simulink library "Contact_Forces_Lib"  (R2025a)
settings: Solver=ode45  StartTime=0.0  StopTime=10.0  RelTol=1e-3  EnableMultiTasking=on
undefined symbols (not defined in the file or in its folder): b_contact, custom_param_1, custom_param_2, Extr_Data_Ring, k_contact, l_cone, length_cylinder, length_tube, mu_kinetic, mu_static, pen_exponent, pen_full_damp_F, rad_s_cone, radius_cylinder, radius_tube, v_thr, X, Y, Z
libraries: nesl_utility x197, sm_lib x115, $bdroot x72, simulink x20, fl_lib x4
(part 9 of 12)

== system Contact_Forces_Lib/2D/Composite Forces/Box to Box Force/BoxB Corners ==
  Circle to Line C1 AC : $bdroot/2D/Circle to Finite Line Force  circle_rad=boxB_contact_rad  line_depth=boxF_h/2  line_length=boxF_l  force_law=Linear  k_contact=k_contact_box2box  b_contact=b_contact_box2box  pen_full_damp_F=pen_full_damp_F_box2box  pen_exponent=pen_exponent_box2box  custom_param_1=1  custom_param_2=1  friction_law=None  mu_kinetic=mu_kinetic_box2box  mu_static=mu_static_box2box  v_thr=v_thr_box2box  vis_on=off  vis_opc_en=0  vis_len_linBz=vis_len_boxFz  vis_len_linBx=vis_len_boxFx  vis_len_cirFz=vis_len_boxBz  vis_len_cirFx=vis_len_boxBx  vis_clr=vis_clr_box2box  vis_opc=vis_opc_box2box
  Circle to Line C1 BD : $bdroot/2D/Circle to Finite Line Force  circle_rad=boxB_contact_rad  line_depth=boxF_l/2  line_length=boxF_h  force_law=Linear  k_contact=k_contact_box2box  b_contact=b_contact_box2box  pen_full_damp_F=pen_full_damp_F_box2box  pen_exponent=pen_exponent_box2box  custom_param_1=1  custom_param_2=1  friction_law=None  mu_kinetic=mu_kinetic_box2box  mu_static=mu_static_box2box  v_thr=v_thr_box2box  vis_on=off  vis_opc_en=0  vis_len_linBz=vis_len_boxFz  vis_len_linBx=vis_len_boxFx  vis_len_cirFz=vis_len_boxBz  vis_len_cirFx=vis_len_boxBx  vis_clr=vis_clr_box2box  vis_opc=vis_opc_box2box
  Circle to Line C2 AC : $bdroot/2D/Circle to Finite Line Force  circle_rad=boxB_contact_rad  line_depth=boxF_h/2  line_length=boxF_l  force_law=Linear  k_contact=k_contact_box2box  b_contact=b_contact_box2box  pen_full_damp_F=pen_full_damp_F_box2box  pen_exponent=pen_exponent_box2box  custom_param_1=1  custom_param_2=1  friction_law=None  mu_kinetic=mu_kinetic_box2box  mu_static=mu_static_box2box  v_thr=v_thr_box2box  vis_on=off  vis_opc_en=0  vis_len_linBz=vis_len_boxFz  vis_len_linBx=vis_len_boxFx  vis_len_cirFz=vis_len_boxBz  vis_len_cirFx=vis_len_boxBx  vis_clr=vis_clr_box2box  vis_opc=vis_opc_box2box
  Circle to Line C2 BD : $bdroot/2D/Circle to Finite Line Force  circle_rad=boxB_contact_rad  line_depth=boxF_l/2  line_length=boxF_h  force_law=Linear  k_contact=k_contact_box2box  b_contact=b_contact_box2box  pen_full_damp_F=pen_full_damp_F_box2box  pen_exponent=pen_exponent_box2box  custom_param_1=1  custom_param_2=1  friction_law=None  mu_kinetic=mu_kinetic_box2box  mu_static=mu_static_box2box  v_thr=v_thr_box2box  vis_on=off  vis_opc_en=0  vis_len_linBz=vis_len_boxFz  vis_len_linBx=vis_len_boxFx  vis_len_cirFz=vis_len_boxBz  vis_len_cirFx=vis_len_boxBx  vis_clr=vis_clr_box2box  vis_opc=vis_opc_box2box
  Circle to Line C3 AC : $bdroot/2D/Circle to Finite Line Force  circle_rad=boxB_contact_rad  line_depth=boxF_h/2  line_length=boxF_l  force_law=Linear  k_contact=k_contact_box2box  b_contact=b_contact_box2box  pen_full_damp_F=pen_full_damp_F_box2box  pen_exponent=pen_exponent_box2box  custom_param_1=1  custom_param_2=1  friction_law=None  mu_kinetic=mu_kinetic_box2box  mu_static=mu_static_box2box  v_thr=v_thr_box2box  vis_on=off  vis_opc_en=0  vis_len_linBz=vis_len_boxFz  vis_len_linBx=vis_len_boxFx  vis_len_cirFz=vis_len_boxBz  vis_len_cirFx=vis_len_boxBx  vis_clr=vis_clr_box2box  vis_opc=vis_opc_box2box
  Circle to Line C3 BD : $bdroot/2D/Circle to Finite Line Force  circle_rad=boxB_contact_rad  line_depth=boxF_l/2  line_length=boxF_h  force_law=Linear  k_contact=k_contact_box2box  b_contact=b_contact_box2box  pen_full_damp_F=pen_full_damp_F_box2box  pen_exponent=pen_exponent_box2box  custom_param_1=1  custom_param_2=1  friction_law=None  mu_kinetic=mu_kinetic_box2box  mu_static=mu_static_box2box  v_thr=v_thr_box2box  vis_on=off  vis_opc_en=0  vis_len_linBz=vis_len_boxFz  vis_len_linBx=vis_len_boxFx  vis_len_cirFz=vis_len_boxBz  vis_len_cirFx=vis_len_boxBx  vis_clr=vis_clr_box2box  vis_opc=vis_opc_box2box
  Circle to Line C4 AC : $bdroot/2D/Circle to Finite Line Force  circle_rad=boxB_contact_rad  line_depth=boxF_h/2  line_length=boxF_l  force_law=Linear  k_contact=k_contact_box2box  b_contact=b_contact_box2box  pen_full_damp_F=pen_full_damp_F_box2box  pen_exponent=pen_exponent_box2box  custom_param_1=1  custom_param_2=1  friction_law=None  mu_kinetic=mu_kinetic_box2box  mu_static=mu_static_box2box  v_thr=v_thr_box2box  vis_on=off  vis_opc_en=0  vis_len_linBz=vis_len_boxFz  vis_len_linBx=vis_len_boxFx  vis_len_cirFz=vis_len_boxBz  vis_len_cirFx=vis_len_boxBx  vis_clr=vis_clr_box2box  vis_opc=vis_opc_box2box
  Circle to Line C4 BD : $bdroot/2D/Circle to Finite Line Force  circle_rad=boxB_contact_rad  line_depth=boxF_l/2  line_length=boxF_h  force_law=Linear  k_contact=k_contact_box2box  b_contact=b_contact_box2box  pen_full_damp_F=pen_full_damp_F_box2box  pen_exponent=pen_exponent_box2box  custom_param_1=1  custom_param_2=1  friction_law=None  mu_kinetic=mu_kinetic_box2box  mu_static=mu_static_box2box  v_thr=v_thr_box2box  vis_on=off  vis_opc_en=0  vis_len_linBz=vis_len_boxFz  vis_len_linBx=vis_len_boxFx  vis_len_cirFz=vis_len_boxBz  vis_len_cirFx=vis_len_boxBx  vis_clr=vis_clr_box2box  vis_opc=vis_opc_box2box
  Forces : Subsystem
  Transform  C1 : sm_lib/Frames and Transforms/Rigid Transform  RotationMethod=None  FollAlignAxisA=+X  BaseAlignAxisA=+Y  FollAlignAxisB=+Y  BaseAlignAxisB=+Z  RotationStandardAxis=+Z  RotationAngle=0  RotationAngleUnits=deg  RotationArbitraryAxis=[0 0 1]  RotationSequenceAxes=FollowerAxes  RotationSequence=XYX  RotationSequenceAngles=[0 0 0]  RotationSequenceAnglesUnits=deg  RotationMatrix=[1 0 0; 0 1 0; 0 0 1]  Quaternion=[1 0 0 0]  TranslationMethod=Cartesian  TranslationCartesianOffset=[-(boxB_h/2-boxB_contact_rad) -(boxB_l/2-boxB_contact_rad) 0]  TranslationCartesianOffsetUnits=m  TranslationStandardAxis=+Y  TranslationStandardOffset=0.1  TranslationStandardOffsetUnits=m  TranslationROffset=0  TranslationROffsetUnits=m  TranslationThetaOffset=0  TranslationThetaOffsetUnits=deg  TranslationZOffset=0  TranslationZOffsetUnits=m
  Transform  C2 : sm_lib/Frames and Transforms/Rigid Transform  RotationMethod=None  FollAlignAxisA=+X  BaseAlignAxisA=+Y  FollAlignAxisB=+Y  BaseAlignAxisB=+Z  RotationStandardAxis=+Z  RotationAngle=0  RotationAngleUnits=deg  RotationArbitraryAxis=[0 0 1]  RotationSequenceAxes=FollowerAxes  RotationSequence=XYX  RotationSequenceAngles=[0 0 0]  RotationSequenceAnglesUnits=deg  RotationMatrix=[1 0 0; 0 1 0; 0 0 1]  Quaternion=[1 0 0 0]  TranslationMethod=Cartesian  TranslationCartesianOffset=[-(boxB_h/2-boxB_contact_rad) (boxB_l/2-boxB_contact_rad) 0]  TranslationCartesianOffsetUnits=m  TranslationStandardAxis=+Y  TranslationStandardOffset=0.1  TranslationStandardOffsetUnits=m  TranslationROffset=0  TranslationROffsetUnits=m  TranslationThetaOffset=0  TranslationThetaOffsetUnits=deg  TranslationZOffset=0  TranslationZOffsetUnits=m
  Transform  C3 : sm_lib/Frames and Transforms/Rigid Transform  RotationMethod=None  FollAlignAxisA=+X  BaseAlignAxisA=+Y  FollAlignAxisB=+Y  BaseAlignAxisB=+Z  RotationStandardAxis=+Z  RotationAngle=0  RotationAngleUnits=deg  RotationArbitraryAxis=[0 0 1]  RotationSequenceAxes=FollowerAxes  RotationSequence=XYX  RotationSequenceAngles=[0 0 0]  RotationSequenceAnglesUnits=deg  RotationMatrix=[1 0 0; 0 1 0; 0 0 1]  Quaternion=[1 0 0 0]  TranslationMethod=Cartesian  TranslationCartesianOffset=[(boxB_h/2-boxB_contact_rad) (boxB_l/2-boxB_contact_rad) 0]  TranslationCartesianOffsetUnits=m  TranslationStandardAxis=+Y  TranslationStandardOffset=0.1  TranslationStandardOffsetUnits=m  TranslationROffset=0  TranslationROffsetUnits=m  TranslationThetaOffset=0  TranslationThetaOffsetUnits=deg  TranslationZOffset=0  TranslationZOffsetUnits=m
  Transform  C4 : sm_lib/Frames and Transforms/Rigid Transform  RotationMethod=None  FollAlignAxisA=+X  BaseAlignAxisA=+Y  FollAlignAxisB=+Y  BaseAlignAxisB=+Z  RotationStandardAxis=+Z  RotationAngle=0  RotationAngleUnits=deg  RotationArbitraryAxis=[0 0 1]  RotationSequenceAxes=FollowerAxes  RotationSequence=XYX  RotationSequenceAngles=[0 0 0]  RotationSequenceAnglesUnits=deg  RotationMatrix=[1 0 0; 0 1 0; 0 0 1]  Quaternion=[1 0 0 0]  TranslationMethod=Cartesian  TranslationCartesianOffset=[(boxB_h/2-boxB_contact_rad) -(boxB_l/2-boxB_contact_rad) 0]  TranslationCartesianOffsetUnits=m  TranslationStandardAxis=+Y  TranslationStandardOffset=0.1  TranslationStandardOffsetUnits=m  TranslationROffset=0  TranslationROffsetUnits=m  TranslationThetaOffset=0  TranslationThetaOffsetUnits=deg  TranslationZOffset=0  TranslationZOffsetUnits=m
  Transform BD : sm_lib/Frames and Transforms/Rigid Transform  RotationMethod=StandardAxis  FollAlignAxisA=+X  BaseAlignAxisA=+Y  FollAlignAxisB=+Y  BaseAlignAxisB=+Z  RotationStandardAxis=+Z  RotationAngle=90  RotationAngleUnits=deg  RotationArbitraryAxis=[0 0 1]  RotationSequenceAxes=FollowerAxes  RotationSequence=XYX  RotationSequenceAngles=[0 0 0]  RotationSequenceAnglesUnits=deg  RotationMatrix=[1 0 0; 0 1 0; 0 0 1]  Quaternion=[1 0 0 0]  TranslationMethod=None  TranslationCartesianOffset=[0 0 0]  TranslationCartesianOffsetUnits=m  TranslationStandardAxis=+Y  TranslationStandardOffset=0.1  TranslationStandardOffsetUnits=m  TranslationROffset=0  TranslationROffsetUnits=m  TranslationThetaOffset=0  TranslationThetaOffsetUnits=deg  TranslationZOffset=0  TranslationZOffsetUnits=m
  BoxB : PMIOPort  Side=Left
  BoxF : PMIOPort  Port=2  Side=Right
  wires:
  Circle to Line C4 BD/1 -> Forces/8(4BD)
  Circle to Line C2 BD/1 -> Forces/4(2BD)
  Circle to Line C3 BD/1 -> Forces/6(3BD)
  Circle to Line C1 AC/1 -> Forces/1(1AC)
  Circle to Line C3 AC/1 -> Forces/5(3AC)
  Circle to Line C4 AC/1 -> Forces/7(4AC)
  Circle to Line C2 AC/1 -> Forces/3(2AC)
  Circle to Line C1 BD/1 -> Forces/2(1BD)
  connections:
  Circle to Line C3 BD/RConn1 -- Circle to Line C4 BD/RConn1 -- Circle to Line C2 BD/RConn1 -- Transform BD/RConn1 -- Circle to Line C1 BD/RConn1
  Circle to Line C1 AC/LConn1 -- Circle to Line C1 BD/LConn1 -- Transform  C1/RConn1
  Transform BD/LConn1 -- BoxF/RConn1 -- Circle to Line C3 AC/RConn1 -- Circle to Line C4 AC/RConn1 -- Circle to Line C2 AC/RConn1 -- Circle to Line C1 AC/RConn1
  Transform  C3/LConn1 -- Transform  C4/LConn1 -- BoxB/RConn1 -- Transform  C1/LConn1 -- Transform  C2/LConn1
  Circle to Line C3 AC/LConn1 -- Circle to Line C3 BD/LConn1 -- Transform  C3/RConn1
  Circle to Line C4 AC/LConn1 -- Circle to Line C4 BD/LConn1 -- Transform  C4/RConn1
  Circle to Line C2 AC/LConn1 -- Circle to Line C2 BD/LConn1 -- Transform  C2/RConn1

== system Contact_Forces_Lib/2D/Composite Forces/Box to Box Force/BoxF Corners ==
  Circle to Line C1 AC : $bdroot/2D/Circle to Finite Line Force  circle_rad=boxF_contact_rad  line_depth=boxB_h/2  line_length=boxB_l  force_law=Linear  k_contact=k_contact_box2box  b_contact=b_contact_box2box  pen_full_damp_F=pen_full_damp_F_box2box  pen_exponent=pen_exponent_box2box  custom_param_1=1  custom_param_2=1  friction_law=None  mu_kinetic=mu_kinetic_box2box  mu_static=mu_static_box2box  v_thr=v_thr_box2box  vis_on=off  vis_opc_en=0  vis_len_linBz=vis_len_boxBz  vis_len_linBx=vis_len_boxBx  vis_len_cirFz=vis_len_boxFz  vis_len_cirFx=vis_len_boxFx  vis_clr=vis_clr_box2box  vis_opc=vis_opc_box2box
  Circle to Line C1 BD : $bdroot/2D/Circle to Finite Line Force  circle_rad=boxF_contact_rad  line_depth=boxB_l/2  line_length=boxB_h  force_law=Linear  k_contact=k_contact_box2box  b_contact=b_contact_box2box  pen_full_damp_F=pen_full_damp_F_box2box  pen_exponent=pen_exponent_box2box  custom_param_1=1  custom_param_2=1  friction_law=None  mu_kinetic=mu_kinetic_box2box  mu_static=mu_static_box2box  v_thr=v_thr_box2box  vis_on=off  vis_opc_en=0  vis_len_linBz=vis_len_boxBz  vis_len_linBx=vis_len_boxBx  vis_len_cirFz=vis_len_boxFz  vis_len_cirFx=vis_len_boxFx  vis_clr=vis_clr_box2box  vis_opc=vis_opc_box2box
  Circle to Line C2 AC : $bdroot/2D/Circle to Finite Line Force  circle_rad=boxF_contact_rad  line_depth=boxB_h/2  line_length=boxB_l  force_law=Linear  k_contact=k_contact_box2box  b_contact=b_contact_box2box  pen_full_damp_F=pen_full_damp_F_box2box  pen_exponent=pen_exponent_box2box  custom_param_1=1  custom_param_2=1  friction_law=None  mu_kinetic=mu_kinetic_box2box  mu_static=mu_static_box2box  v_thr=v_thr_box2box  vis_on=off  vis_opc_en=0  vis_len_linBz=vis_len_boxBz  vis_len_linBx=vis_len_boxBx  vis_len_cirFz=vis_len_boxFz  vis_len_cirFx=vis_len_boxFx  vis_clr=vis_clr_box2box  vis_opc=vis_opc_box2box
  Circle to Line C2 BD : $bdroot/2D/Circle to Finite Line Force  circle_rad=boxF_contact_rad  line_depth=boxB_l/2  line_length=boxB_h  force_law=Linear  k_contact=k_contact_box2box  b_contact=b_contact_box2box  pen_full_damp_F=pen_full_damp_F_box2box  pen_exponent=pen_exponent_box2box  custom_param_1=1  custom_param_2=1  friction_law=None  mu_kinetic=mu_kinetic_box2box  mu_static=mu_static_box2box  v_thr=v_thr_box2box  vis_on=off  vis_opc_en=0  vis_len_linBz=vis_len_boxBz  vis_len_linBx=vis_len_boxBx  vis_len_cirFz=vis_len_boxFz  vis_len_cirFx=vis_len_boxFx  vis_clr=vis_clr_box2box  vis_opc=vis_opc_box2box
  Circle to Line C3 AC : $bdroot/2D/Circle to Finite Line Force  circle_rad=boxF_contact_rad  line_depth=boxB_h/2  line_length=boxB_l  force_law=Linear  k_contact=k_contact_box2box  b_contact=b_contact_box2box  pen_full_damp_F=pen_full_damp_F_box2box  pen_exponent=pen_exponent_box2box  custom_param_1=1  custom_param_2=1  friction_law=None  mu_kinetic=mu_kinetic_box2box  mu_static=mu_static_box2box  v_thr=v_thr_box2box  vis_on=off  vis_opc_en=0  vis_len_linBz=vis_len_boxBz  vis_len_linBx=vis_len_boxBx  vis_len_cirFz=vis_len_boxFz  vis_len_cirFx=vis_len_boxFx  vis_clr=vis_clr_box2box  vis_opc=vis_opc_box2box
  Circle to Line C3 BD : $bdroot/2D/Circle to Finite Line Force  circle_rad=boxF_contact_rad  line_depth=boxB_l/2  line_length=boxB_h  force_law=Linear  k_contact=k_contact_box2box  b_contact=b_contact_box2box  pen_full_damp_F=pen_full_damp_F_box2box  pen_exponent=pen_exponent_box2box  custom_param_1=1  custom_param_2=1  friction_law=None  mu_kinetic=mu_kinetic_box2box  mu_static=mu_static_box2box  v_thr=v_thr_box2box  vis_on=off  vis_opc_en=0  vis_len_linBz=vis_len_boxBz  vis_len_linBx=vis_len_boxBx  vis_len_cirFz=vis_len_boxFz  vis_len_cirFx=vis_len_boxFx  vis_clr=vis_clr_box2box  vis_opc=vis_opc_box2box
  Circle to Line C4 AC : $bdroot/2D/Circle to Finite Line Force  circle_rad=boxF_contact_rad  line_depth=boxB_h/2  line_length=boxB_l  force_law=Linear  k_contact=k_contact_box2box  b_contact=b_contact_box2box  pen_full_damp_F=pen_full_damp_F_box2box  pen_exponent=pen_exponent_box2box  custom_param_1=1  custom_param_2=1  friction_law=None  mu_kinetic=mu_kinetic_box2box  mu_static=mu_static_box2box  v_thr=v_thr_box2box  vis_on=off  vis_opc_en=0  vis_len_linBz=vis_len_boxBz  vis_len_linBx=vis_len_boxBx  vis_len_cirFz=vis_len_boxFz  vis_len_cirFx=vis_len_boxFx  vis_clr=vis_clr_box2box  vis_opc=vis_opc_box2box
  Circle to Line C4 BD : $bdroot/2D/Circle to Finite Line Force  circle_rad=boxF_contact_rad  line_depth=boxB_l/2  line_length=boxB_h  force_law=Linear  k_contact=k_contact_box2box  b_contact=b_contact_box2box  pen_full_damp_F=pen_full_damp_F_box2box  pen_exponent=pen_exponent_box2box  custom_param_1=1  custom_param_2=1  friction_law=None  mu_kinetic=mu_kinetic_box2box  mu_static=mu_static_box2box  v_thr=v_thr_box2box  vis_on=off  vis_opc_en=0  vis_len_linBz=vis_len_boxBz  vis_len_linBx=vis_len_boxBx  vis_len_cirFz=vis_len_boxFz  vis_len_cirFx=vis_len_boxFx  vis_clr=vis_clr_box2box  vis_opc=vis_opc_box2box
  Forces : Subsystem
  Transform BD : sm_lib/Frames and Transforms/Rigid Transform  RotationMethod=StandardAxis  FollAlignAxisA=+X  BaseAlignAxisA=+Y  FollAlignAxisB=+Y  BaseAlignAxisB=+Z  RotationStandardAxis=+Z  RotationAngle=90  RotationAngleUnits=deg  RotationArbitraryAxis=[0 0 1]  RotationSequenceAxes=FollowerAxes  RotationSequence=XYX  RotationSequenceAngles=[0 0 0]  RotationSequenceAnglesUnits=deg  RotationMatrix=[1 0 0; 0 1 0; 0 0 1]  Quaternion=[1 0 0 0]  TranslationMethod=None  TranslationCartesianOffset=[0 0 0]  TranslationCartesianOffsetUnits=m  TranslationStandardAxis=+Y  TranslationStandardOffset=0.1  TranslationStandardOffsetUnits=m  TranslationROffset=0  TranslationROffsetUnits=m  TranslationThetaOffset=0  TranslationThetaOffsetUnits=deg  TranslationZOffset=0  TranslationZOffsetUnits=m
  Transform C1 : sm_lib/Frames and Transforms/Rigid Transform  RotationMethod=None  FollAlignAxisA=+X  BaseAlignAxisA=+Y  FollAlignAxisB=+Y  BaseAlignAxisB=+Z  RotationStandardAxis=+Z  RotationAngle=0  RotationAngleUnits=deg  RotationArbitraryAxis=[0 0 1]  RotationSequenceAxes=FollowerAxes  RotationSequence=XYX  RotationSequenceAngles=[0 0 0]  RotationSequenceAnglesUnits=deg  RotationMatrix=[1 0 0; 0 1 0; 0 0 1]  Quaternion=[1 0 0 0]  TranslationMethod=Cartesian  TranslationCartesianOffset=[-(boxF_h/2-boxF_contact_rad) -(boxF_l/2-boxF_contact_rad) 0]  TranslationCartesianOffsetUnits=m  TranslationStandardAxis=+Y  TranslationStandardOffset=0.1  TranslationStandardOffsetUnits=m  TranslationROffset=0  TranslationROffsetUnits=m  TranslationThetaOffset=0  TranslationThetaOffsetUnits=deg  TranslationZOffset=0  TranslationZOffsetUnits=m
  Transform C2 : sm_lib/Frames and Transforms/Rigid Transform  RotationMethod=None  FollAlignAxisA=+X  BaseAlignAxisA=+Y  FollAlignAxisB=+Y  BaseAlignAxisB=+Z  RotationStandardAxis=+Z  RotationAngle=0  RotationAngleUnits=deg  RotationArbitraryAxis=[0 0 1]  RotationSequenceAxes=FollowerAxes  RotationSequence=XYX  RotationSequenceAngles=[0 0 0]  RotationSequenceAnglesUnits=deg  RotationMatrix=[1 0 0; 0 1 0; 0 0 1]  Quaternion=[1 0 0 0]  TranslationMethod=Cartesian  TranslationCartesianOffset=[-(boxF_h/2-boxF_contact_rad) (boxF_l/2-boxF_contact_rad) 0]  TranslationCartesianOffsetUnits=m  TranslationStandardAxis=+Y  TranslationStandardOffset=0.1  TranslationStandardOffsetUnits=m  TranslationROffset=0  TranslationROffsetUnits=m  TranslationThetaOffset=0  TranslationThetaOffsetUnits=deg  TranslationZOffset=0  TranslationZOffsetUnits=m
  Transform C3 : sm_lib/Frames and Transforms/Rigid Transform  RotationMethod=None  FollAlignAxisA=+X  BaseAlignAxisA=+Y  FollAlignAxisB=+Y  BaseAlignAxisB=+Z  RotationStandardAxis=+Z  RotationAngle=0  RotationAngleUnits=deg  RotationArbitraryAxis=[0 0 1]  RotationSequenceAxes=FollowerAxes  RotationSequence=XYX  RotationSequenceAngles=[0 0 0]  RotationSequenceAnglesUnits=deg  RotationMatrix=[1 0 0; 0 1 0; 0 0 1]  Quaternion=[1 0 0 0]  TranslationMethod=Cartesian  TranslationCartesianOffset=[(boxF_h/2-boxF_contact_rad) (boxF_l/2-boxF_contact_rad) 0]  TranslationCartesianOffsetUnits=m  TranslationStandardAxis=+Y  TranslationStandardOffset=0.1  TranslationStandardOffsetUnits=m  TranslationROffset=0  TranslationROffsetUnits=m  TranslationThetaOffset=0  TranslationThetaOffsetUnits=deg  TranslationZOffset=0  TranslationZOffsetUnits=m
  Transform C4 : sm_lib/Frames and Transforms/Rigid Transform  RotationMethod=None  FollAlignAxisA=+X  BaseAlignAxisA=+Y  FollAlignAxisB=+Y  BaseAlignAxisB=+Z  RotationStandardAxis=+Z  RotationAngle=0  RotationAngleUnits=deg  RotationArbitraryAxis=[0 0 1]  RotationSequenceAxes=FollowerAxes  RotationSequence=XYX  RotationSequenceAngles=[0 0 0]  RotationSequenceAnglesUnits=deg  RotationMatrix=[1 0 0; 0 1 0; 0 0 1]  Quaternion=[1 0 0 0]  TranslationMethod=Cartesian  TranslationCartesianOffset=[(boxF_h/2-boxF_contact_rad) -(boxF_l/2-boxF_contact_rad) 0]  TranslationCartesianOffsetUnits=m  TranslationStandardAxis=+Y  TranslationStandardOffset=0.1  TranslationStandardOffsetUnits=m  TranslationROffset=0  TranslationROffsetUnits=m  TranslationThetaOffset=0  TranslationThetaOffsetUnits=deg  TranslationZOffset=0  TranslationZOffsetUnits=m
  BoxB : PMIOPort  Side=Left
  BoxF : PMIOPort  Port=2  Side=Right
  wires:
  Circle to Line C4 AC/1 -> Forces/7(4AC)
  Circle to Line C1 BD/1 -> Forces/2(1BD)
  Circle to Line C2 AC/1 -> Forces/3(2AC)
  Circle to Line C3 BD/1 -> Forces/6(3BD)
  Circle to Line C4 BD/1 -> Forces/8(4BD)
  Circle to Line C2 BD/1 -> Forces/4(2BD)
  Circle to Line C3 AC/1 -> Forces/5(3AC)
  Circle to Line C1 AC/1 -> Forces/1(1AC)
  connections:
  Circle to Line C1 BD/RConn1 -- Transform BD/RConn1 -- Circle to Line C3 BD/RConn1 -- Circle to Line C4 BD/RConn1 -- Circle to Line C2 BD/RConn1
  Circle to Line C2 AC/LConn1 -- Circle to Line C2 BD/LConn1 -- Transform C2/RConn1
  Circle to Line C3 AC/LConn1 -- Circle to Line C3 BD/LConn1 -- Transform C3/RConn1
  Transform C3/LConn1 -- Transform C4/LConn1 -- Transform C1/LConn1 -- Transform C2/LConn1 -- BoxF/RConn1
  Circle to Line C4 AC/LConn1 -- Circle to Line C4 BD/LConn1 -- Transform C4/RConn1
  Transform BD/LConn1 -- Circle to Line C1 AC/RConn1 -- Circle to Line C2 AC/RConn1 -- Circle to Line C3 AC/RConn1 -- Circle to Line C4 AC/RConn1 -- BoxB/RConn1
  Circle to Line C1 BD/LConn1 -- Circle to Line C1 AC/LConn1 -- Transform C1/RConn1

== system Contact_Forces_Lib/3D/Prototype/Cone in Ring Force/Enable ==
  z : Inport
  R : Inport  Port=2
  Add1 : Sum  Inputs=+-
  Add3 : Sum  Inputs=+-
  Constant1 : Constant  Value=l_cyl/2+lc
  Constant2 : Constant  Value=l_tube/2
  Constant4 : Constant  Value=l_cyl/2
  Constant5 : Constant  Value=l_tube/2
  Logical Operator : Logic  AllPortsSameDT=off  OutDataTypeStr=boolean
  Product : Product
  Product1 : Product
  Relational Operator1 : RelationalOperator  OutDataTypeStr=boolean  ZeroCross=off  InputSameDT=off
  Relational Operator2 : RelationalOperator  Operator=<=  OutDataTypeStr=boolean  ZeroCross=off  InputSameDT=off
  Selector : Selector  NumberOfDimensions=2  InputPortWidth=3  IndexOptions=Index vector (dialog),Index vector (dialog)  Indices=3,3  OutputSizes=1,1
  Enable : Outport  VectorParamsAs1DForOutWhenUnconnected=off
  wires:
  Constant5/1 -> Relational Operator1/2
  Add3/1 -> Relational Operator1/1
  Relational Operator1/1 -> Logical Operator/1
  Constant2/1 -> Relational Operator2/2
  z/1 -> Add1/1, Add3/1
  Add1/1 -> Relational Operator2/1
  Relational Operator2/1 -> Logical Operator/2
  Logical Operator/1 -> Enable/1
  R/1 -> Selector/1
  Constant4/1 -> Product/1
  Product/1 -> Add3/2
  Selector/1 -> Product1/1, Product/2  "r33"
  Constant1/1 -> Product1/2
  Product1/1 -> Add1/2

== system Contact_Forces_Lib/3D/Prototype/Cone in Ring Force/If Action Subsystem ==
  Action Port : ActionPort
  Constant : Constant  Value=[0 0 0]  SampleTime=0
  F : Outport  VectorParamsAs1DForOutWhenUnconnected=off
  T : Outport  Port=2  VectorParamsAs1DForOutWhenUnconnected=off
  wires:
  Constant/1 -> T/1, F/1

== system Contact_Forces_Lib/3D/Prototype/Cone in Ring Force/Point of Contact calc ==
  note: Xb = r11*r*cos(th) + r12*r*sin(th) +r13*z + Xc;
      | Yb = r21*r*cos(th) + r22*r*sin(th) +r23*z + Yc;
  R : Inport
  x : Inport  Port=2
  y : Inport  Port=3
  z : Inport  Port=4
  Action Port : ActionPort
  Constant1 : Constant  Value=[0:2*pi/n:2*pi]
  Cross Product : Subsystem
  Demux : Demux  Outputs=3
  Demux1 : Demux  Outputs=3
  Demux2 : Demux  Outputs=3
  Force Calc : Subsystem
  Mux : Mux  Inputs=3
  R1 : InportShadow
  Selector : Selector  NumberOfDimensions=2  InputPortWidth=3  IndexOptions=Index vector (dialog),Index vector (dialog)  Indices=1,[1:3]  OutputSizes=1,1
  Selector1 : Selector  NumberOfDimensions=2  InputPortWidth=3  IndexOptions=Index vector (dialog),Index vector (dialog)  Indices=2,[1:3]  OutputSizes=1,1
  Selector2 : Selector  NumberOfDimensions=2  InputPortWidth=3  IndexOptions=Index vector (dialog),Index vector (dialog)  Indices=3,[1:3]  OutputSizes=1,1
  r calc : Subsystem
  x calc : Subsystem
  y calc : Subsystem
  z calc : Subsystem
  F : Outport  VectorParamsAs1DForOutWhenUnconnected=off
  T : Outport  Port=2  VectorParamsAs1DForOutWhenUnconnected=off
  wires:
  R/1 -> Selector2/1, Selector1/1, Selector/1
  Selector/1 -> Demux/1
  Selector1/1 -> Demux1/1
  Selector2/1 -> Demux2/1
  Demux2/1 -> z calc/1(r31)  "r31"
  Demux2/2 -> z calc/2(r32)  "r32"
  Demux2/3 -> z calc/3(r33)  "r33"
  z/1 -> z calc/4(zc)
  Constant1/1 -> Force Calc/5(th), x calc/5(th), y calc/5(th), z calc/5(th)
  Demux/1 -> x calc/1(r11)
  Demux/2 -> x calc/2(r12)
  Demux/3 -> x calc/3(r13)
  x/1 -> x calc/4(xc)
  z calc/1(z) -> Force Calc/4(z), y calc/6(z), x calc/6(z), r calc/1(z)
  Demux1/1 -> y calc/1(r21)
  Demux1/2 -> y calc/2(r22)
  Demux1/3 -> y calc/3(r23)
  y/1 -> y calc/4(yc)
  x calc/1(x) -> Force Calc/1(x)
  y calc/1(y) -> Force Calc/2(y)
  Force Calc/1(Fx) -> Mux/1
  Force Calc/2(Fy) -> Mux/2
  r calc/1(r) -> Force Calc/3(r), x calc/7(r), y calc/7(r)
  Force Calc/3(Fz) -> Mux/3
  Mux/1 -> Cross Product/2(In2), F/1
  Force Calc/4(pc) -> Cross Product/1(In1)
  Cross Product/1(Out1) -> T/1

== system Contact_Forces_Lib/3D/Prototype/Cylinder In Ring Force/Enable ==
  z : Inport
  R : Inport  Port=2
  Abs : Abs  ZeroCross=off  SaturateOnIntegerOverflow=off
  Add2 : Sum
  Add3 : Sum  Inputs=+-
  Constant2 : Constant  Value=l_tube/2
  Constant3 : Constant  Value=l_cyl/2
  Constant4 : Constant  Value=l_cyl/2
  Constant5 : Constant  Value=l_tube/2
  Logical Operator : Logic  AllPortsSameDT=off  OutDataTypeStr=boolean
  Product : Product
  Product1 : Product
  Relational Operator : RelationalOperator  OutDataTypeStr=boolean  ZeroCross=off  InputSameDT=off
  Relational Operator1 : RelationalOperator  Operator=<=  OutDataTypeStr=boolean  ZeroCross=off  InputSameDT=off
  Selector : Selector  NumberOfDimensions=2  InputPortWidth=3  IndexOptions=Index vector (dialog),Index vector (dialog)  Indices=3,3  OutputSizes=1,1
  Enable : Outport  VectorParamsAs1DForOutWhenUnconnected=off
  wires:
  z/1 -> Abs/1
  Logical Operator/1 -> Enable/1
  Constant5/1 -> Relational Operator1/2
  Constant2/1 -> Relational Operator/2
  Relational Operator/1 -> Logical Operator/1
  Abs/1 -> Add3/1, Add2/2
  Relational Operator1/1 -> Logical Operator/2
  Add2/1 -> Relational Operator/1
  Add3/1 -> Relational Operator1/1
  R/1 -> Selector/1
  Selector/1 -> Product1/2, Product/1  "r33"
  Product/1 -> Add3/2
  Constant4/1 -> Product/2
  Product1/1 -> Add2/1
  Constant3/1 -> Product1/1

== system Contact_Forces_Lib/3D/Prototype/Cylinder In Ring Force/If Action Subsystem ==
  Action Port : ActionPort
  Constant : Constant  Value=[0 0 0]  SampleTime=0
  F : Outport  VectorParamsAs1DForOutWhenUnconnected=off
  T : Outport  Port=2  VectorParamsAs1DForOutWhenUnconnected=off
  wires:
  Constant/1 -> T/1, F/1

== system Contact_Forces_Lib/3D/Prototype/Cylinder In Ring Force/Point of Contact calc ==
  note: z = (L/2 - r31*r*cos(th) - r32*r*sin(th) - Zc)/r33;
      | Xb = r11*r*cos(th) + r12*r*sin(th) +r13*z + Xc;
      | Yb = r21*r*cos(th) + r22*r*sin(th) +r23*z + Yc;
  R : Inport
  x : Inport  Port=2
  y : Inport  Port=3
  z : Inport  Port=4
  vz : Inport  Port=5
  Action Port : ActionPort
  Constant1 : Constant  Value=[0:2*pi/n:2*pi]
  Cross Product : Subsystem
  Demux : Demux  Outputs=3
  Demux1 : Demux  Outputs=3
  Demux2 : Demux  Outputs=3
  Divide : Product  Inputs=/*  Multiplication=Matrix(*)
  Force Calc : Subsystem
  Mux : Mux  Inputs=3
  R1 : InportShadow
  Selector : Selector  NumberOfDimensions=2  InputPortWidth=3  IndexOptions=Index vector (dialog),Index vector (dialog)  Indices=1,[1:3]  OutputSizes=1,1
  Selector1 : Selector  NumberOfDimensions=2  InputPortWidth=3  IndexOptions=Index vector (dialog),Index vector (dialog)  Indices=2,[1:3]  OutputSizes=1,1
  Selector2 : Selector  NumberOfDimensions=2  InputPortWidth=3  IndexOptions=Index vector (dialog),Index vector (dialog)  Indices=3,[1:3]  OutputSizes=1,1
  x calc : Subsystem
  y calc : Subsystem
  z calc : Subsystem
  F : Outport  VectorParamsAs1DForOutWhenUnconnected=off
  T : Outport  Port=2  VectorParamsAs1DForOutWhenUnconnected=off
  pen : Outport  Port=3  VectorParamsAs1DForOutWhenUnconnected=off
  wires:
  R/1 -> Selector2/1, Selector1/1, Selector/1
  Selector/1 -> Demux/1
  Selector1/1 -> Demux1/1
  Selector2/1 -> Demux2/1
  Demux2/1 -> z calc/1(r31)  "r31"
  Demux2/2 -> z calc/2(r32)  "r32"
  Demux2/3 -> z calc/3(r33)  "r33"
  z/1 -> z calc/4(zc)
  Constant1/1 -> Force Calc/5(th), y calc/5(th), x calc/5(th), z calc/5(th)
  Demux/1 -> x calc/1(r11)
  Demux/2 -> x calc/2(r12)
  Demux/3 -> x calc/3(r13)
  x/1 -> x calc/4(xc)
  z calc/1(z) -> Force Calc/4(z), y calc/6(z), x calc/6(z)
  Demux1/1 -> y calc/1(r21)
  Demux1/2 -> y calc/2(r22)
  Demux1/3 -> y calc/3(r23)
  y/1 -> y calc/4(yc)
  x calc/1(x) -> Force Calc/1(x)
  y calc/1(y) -> Force Calc/2(y)
  R1/1 -> Divide/1
  Force Calc/1(Fx) -> Mux/1
  Force Calc/2(Fy) -> Mux/2
  Mux/1 -> Divide/2
  Divide/1 -> Cross Product/2(In2), F/1
  Force Calc/3(Fz) -> Mux/3
  Force Calc/4(pc) -> Cross Product/1(In1)
  Cross Product/1(Out1) -> T/1
  vz/1 -> Force Calc/3(v)
  Force Calc/5(maxpen) -> pen/1

== system Contact_Forces_Lib/3D/Sphere in Sphere Force/Ff/Check w or v non zero ==
  w : Inport
  v : Inport  Port=2
  Else : Subsystem  TreatAsAtomicUnit=on
  If : If  NumInputs=2  IfExpression=u1 ~= 0 | u2~=0
  mag v : Subsystem
  mag w : Subsystem
  else v is 0 : Outport  VectorParamsAs1DForOutWhenUnconnected=off
  else uv is 0 : Outport  Port=2  VectorParamsAs1DForOutWhenUnconnected=off
  Use SlipVel : Outport  Port=3  VectorParamsAs1DForOutWhenUnconnected=off
  wires:
  Else/2(vuvect) -> else uv is 0/1
  Else/1(vabs) -> else v is 0/1
  If/2 -> Else/Action
  If/1 -> Use SlipVel/1
  mag w/1(mag) -> If/1
  mag v/1(mag) -> If/2
  v/1 -> mag v/1(vect)
  w/1 -> mag w/1(vect)

== system Contact_Forces_Lib/3D/Sphere in Sphere Force/Ff/SlipVel ==
  w : Inport
  v : Inport  Port=2
  dvect : Inport  Port=3
  Action Port : ActionPort
  Add : Sum
  Add1 : Sum  Inputs=+-
  Add2 : Sum  Inputs=+++
  Cross Product : $bdroot/Math/Cross Product  SystemSampleTime=-1  VariantActivationTime=update diagram  EmptyChoice=off  PassThrough=off  PassThroughVariantControl=(default)  EmptyChoiceVariantControl=(default)  AllowFlexibleInterface=on  Latency=0  AutoFrameSizeCalculation=off
  Demux : Demux  Outputs=3
  Dot Product : DotProduct  OutDataTypeStr=Inherit: Inherit via internal rule
  Fsphere_rad : Gain  Gain=sphF_rad
  Gain : Gain
  If : If  ShowElse=off
  If Action Subsystem : Subsystem  TreatAsAtomicUnit=on
  Math Function : Math  Operator=square  SignedPower=on
  Math Function1 : Math  Operator=square  SignedPower=on
  Math Function2 : Math  Operator=square  SignedPower=on
  Product : Product
  Sqrt : Sqrt
  mag : Subsystem
  vabs : Outport  InitialOutput=0  VectorParamsAs1DForOutWhenUnconnected=off
  vuvect : Outport  Port=2  InitialOutput=0  VectorParamsAs1DForOutWhenUnconnected=off
  wires:
  If Action Subsystem/1(Out1) -> vuvect/1
  If/1 -> If Action Subsystem/Action
  Fsphere_rad/1 -> Cross Product/2
  w/1 -> Cross Product/1
  Cross Product/1 -> Add/1
  v/1 -> Add/2
  dvect/1 -> Gain/1
  Add/1 -> Add1/1, Dot Product/1
  Dot Product/1 -> Product/1
  Product/1 -> Add1/2
  Add1/1 -> Demux/1, mag/1(vect), If Action Subsystem/2(In2)
  Demux/1 -> Math Function/1
  Demux/2 -> Math Function1/1
  Demux/3 -> Math Function2/1
  Math Function/1 -> Add2/1
  Math Function1/1 -> Add2/2
  Math Function2/1 -> Add2/3
  Add2/1 -> Sqrt/1
  Sqrt/1 -> vabs/1
  mag/1(mag) -> If/1, If Action Subsystem/1(In1)
  Gain/1 -> Product/2, Dot Product/2, Fsphere_rad/1

== system Contact_Forces_Lib/3D/Sphere in Sphere Force/Ff/mag ==
  vect : Inport
  Add2 : Sum  Inputs=+++
  Demux : Demux  Outputs=3
  Math Function : Math  Operator=square  SignedPower=on
  Math Function1 : Math  Operator=square  SignedPower=on
  Math Function2 : Math  Operator=square  SignedPower=on
  Sqrt : Sqrt
  mag : Outport  VectorParamsAs1DForOutWhenUnconnected=off
  wires:
  Math Function2/1 -> Add2/3
  Demux/3 -> Math Function2/1
  Sqrt/1 -> mag/1
  Math Function1/1 -> Add2/2
  Math Function/1 -> Add2/1
  Add2/1 -> Sqrt/1
  vect/1 -> Demux/1
  Demux/1 -> Math Function/1
  Demux/2 -> Math Function1/1

== system Contact_Forces_Lib/3D/Sphere to Cone Force/Check Active/Check Active Range ==
  azm : Inport
  " Upper Bound" : simulink/Logic and Bit Operations/Compare To Constant  relop=<=  const=active_angle(2)*pi/180  OutDataTypeStr=boolean  ZeroCross=off
  Logical Operator : Logic  AllPortsSameDT=off  OutDataTypeStr=boolean
  Lower Bound : simulink/Logic and Bit Operations/Compare To Constant  relop=>=  const=active_angle(1)*pi/180  OutDataTypeStr=boolean  ZeroCross=off
  En : Outport  VectorParamsAs1DForOutWhenUnconnected=off
  wires:
  azm/1 -> " Upper Bound"/1, Lower Bound/1
  " Upper Bound"/1 -> Logical Operator/1
  Lower Bound/1 -> Logical Operator/2
  Logical Operator/1 -> En/1

== system Contact_Forces_Lib/3D/Sphere to Cone Force/Check Active/In Tube ==
  z : Inport
  Abs : Abs  ZeroCross=off  SaturateOnIntegerOverflow=off
  Activation limit for contact force : Constant  Value=cone_h/2
  Bias : Bias  Bias=-cone_h/2  SaturateOnIntegerOverflow=off
  Compare To Zero : simulink/Logic and Bit Operations/Compare To Zero  relop=>  OutDataTypeStr=boolean  ZeroCross=off
  Scope : Scope  NumInputPorts=4
      settings: ActiveDisplayYMinimum=-6.25  ActiveDisplayYMaximum=6.25
  Sum : Sum  Inputs=+-
  En : Outport  VectorParamsAs1DForOutWhenUnconnected=off
  wires:
  Bias/1 -> Abs/1, Scope/1
  Abs/1 -> Sum/2, Scope/2
  Compare To Zero/1 -> En/1, Scope/4
  z/1 -> Bias/1
  Activation limit for contact force/1 -> Sum/1
  Sum/1 -> Compare To Zero/1, Scope/3

== system Contact_Forces_Lib/3D/Sphere to Cone Force/Forces/Calculate Penetration ==
  note: Calculates SphF frame to midpoint of Cone wall.
      | Absolute value makes it valid for inside or outside contact.
      | Noting the sign allows us to apply the force correctly
  rad : Inport
  vrad : Inport  Port=2
  z : Inport  Port=3
  vzf : Inport  Port=4
  Abs : Abs  ZeroCross=off  SaturateOnIntegerOverflow=off
  Constant : Constant  Value=radius_sphere+d_cone/2*sinConeTh
  Constant1 : Constant  Value=sinConeTh
  Constant2 : Constant  Value=cosConeTh
  Dead Zone : DeadZone  LowerValue=-inf  UpperValue=0
  Product{,1..5} (6 alike) : Product
  Sign : Signum  ZeroCross=off
  Sum : Sum  Inputs=+-
  Sum1 : Sum  Inputs=+--
  Sum2 : Sum
  radius ring : Constant  Value=r_cone
  sign : Outport  VectorParamsAs1DForOutWhenUnconnected=off
  Pen : Outport  Port=2  VectorParamsAs1DForOutWhenUnconnected=off
  Pen Vel : Outport  Port=3  VectorParamsAs1DForOutWhenUnconnected=off
  wires:
  Product4/1 -> Sum2/1
  Sum2/1 -> Product/2
  Product5/1 -> Sum2/2
  vzf/1 -> Product5/2
  vrad/1 -> Product4/2
  Product2/1 -> Sum1/2
  Product3/1 -> Sum1/3
  Constant2/1 -> Product5/1, Product3/1
  z/1 -> Product3/2
  Constant1/1 -> Product1/2, Product2/1, Product4/1
  Product1/1 -> Sum1/1
  rad/1 -> Product2/2
  radius ring/1 -> Product1/1
  Sum1/1 -> Sign/1, Abs/1
  Abs/1 -> Sum/2
  Sign/1 -> Product/1, sign/1
  Product/1 -> Pen Vel/1
  Sum/1 -> Dead Zone/1
  Constant/1 -> Sum/1
  Dead Zone/1 -> Pen/1

== system Contact_Forces_Lib/3D/Sphere to Cone Force/Forces/Ff ==
  note: Sign of Fn indicates if sphere is inside or outside
  Fn : Inport
  z : Inport  Port=2
  R : Inport  Port=3
  azm : Inport  Port=4
  vazm : Inport  Port=5
  wzf : Inport  Port=6
  Pen : Inport  Port=7
  rad : Inport  Port=8
  vrad : Inport  Port=9
  vzf : Inport  Port=10
  wxf : Inport  Port=11
  wyf : Inport  Port=12
  vazmx : Inport  Port=13
  vazmy : Inport  Port=14
  Friction Law : $bdroot/Friction Law  SystemSampleTime=-1  LabelModeActiveChoice=Stick_Slip_C  VariantActivationTime=update diagram  EmptyChoice=off  PassThrough=off  PassThroughVariantControl=(default)  EmptyChoiceVariantControl=(default)  AllowFlexibleInterface=on  Latency=0  AutoFrameSizeCalculation=off
  Relative vel at CP : Subsystem
  Resolve Ff : Subsystem
  Sign : Signum  ZeroCross=off
  FxSphF : Outport  VectorParamsAs1DForOutWhenUnconnected=off
  FySphF : Outport  Port=2  VectorParamsAs1DForOutWhenUnconnected=off
  FzSphF : Outport  Port=3  VectorParamsAs1DForOutWhenUnconnected=off
  FxConB : Outport  Port=4  VectorParamsAs1DForOutWhenUnconnected=off
  FyConB : Outport  Port=5  VectorParamsAs1DForOutWhenUnconnected=off
  FzConB : Outport  Port=6  VectorParamsAs1DForOutWhenUnconnected=off
  TSphF : Outport  Port=7  VectorParamsAs1DForOutWhenUnconnected=off
  TConB : Outport  Port=8  VectorParamsAs1DForOutWhenUnconnected=off
  Ff : Outport  Port=9  VectorParamsAs1DForOutWhenUnconnected=off
  wires:
  [InOut] -> Resolve Ff/1(InOut)
  [InOut] -> Relative vel at CP/1(InOut)
  vrad/1 -> Relative vel at CP/3(vrad)
  vazmy/1 -> Relative vel at CP/7(vazmy)
  vazmx/1 -> Relative vel at CP/6(vazmx)
  Resolve Ff/7(FzConB) -> FzConB/1
  Resolve Ff/3(FzSphF) -> FzSphF/1
  Relative vel at CP/4(alpha) -> Resolve Ff/7(alpha)
  vzf/1 -> Relative vel at CP/9(vzf)
  R/1 -> Resolve Ff/3(R)
  Pen/1 -> Relative vel at CP/4(Pen)
  Fn/1 -> Sign/1, Friction Law/1  "Fn"
  rad/1 -> Relative vel at CP/2(rad)
  vazm/1 -> Relative vel at CP/5(vazm)
  wzf/1 -> Relative vel at CP/8(wzf)
  Friction Law/1 -> Ff/1, Resolve Ff/2(Ff)  "Ff Abs"
  Resolve Ff/1(FxSphF) -> FxSphF/1
  Resolve Ff/2(FySphF) -> FySphF/1
  Resolve Ff/5(FxConB) -> FxConB/1
  Resolve Ff/6(FyConB) -> FyConB/1
  Resolve Ff/4(TSphF) -> TSphF/1
  Resolve Ff/8(TConB) -> TConB/1
  wxf/1 -> Relative vel at CP/10(wxf)
  wyf/1 -> Relative vel at CP/11(wyf)
  azm/1 -> Relative vel at CP/12(azm), Resolve Ff/8(azm)
  Relative vel at CP/3(rConAxtoCP) -> Resolve Ff/6(rConAxtoCP)
  Relative vel at CP/2(rSphtoCP) -> Resolve Ff/5(rSphtoCP)
  Relative vel at CP/1(vRelAbs) -> Friction Law/2  "vRelAbs"
  z/1 -> Resolve Ff/4(z)
  Sign/1 -> [InOut]  "InOut"

== system Contact_Forces_Lib/3D/Sphere to Cone Force/Forces/Fn ==
  note: Resolve Normal Force in
      | Tube B reference frame
  note: Resolve Normal Force in
      | Sphere F reference frame
  Fn : Inport
  z : Inport  Port=2
  rad : Inport  Port=3
  R : Inport  Port=4
  azm : Inport  Port=5
  Equiv Torques : Subsystem
  Fn in SphF : Subsystem
  Fn in TubB : Subsystem
  FxSphF : Outport  VectorParamsAs1DForOutWhenUnconnected=off
  FySphF : Outport  Port=2  VectorParamsAs1DForOutWhenUnconnected=off
  FZSphF : Outport  Port=3  VectorParamsAs1DForOutWhenUnconnected=off
  FxConB : Outport  Port=4  VectorParamsAs1DForOutWhenUnconnected=off
  FyConB : Outport  Port=5  VectorParamsAs1DForOutWhenUnconnected=off
  FzConB : Outport  Port=6  VectorParamsAs1DForOutWhenUnconnected=off
  TxConB : Outport  Port=7  VectorParamsAs1DForOutWhenUnconnected=off
  TyConB : Outport  Port=8  VectorParamsAs1DForOutWhenUnconnected=off
  wires:
  Equiv Torques/2(TyConB) -> TyConB/1
  Equiv Torques/1(TxConB) -> TxConB/1
  z/1 -> Equiv Torques/6(z)
  rad/1 -> Equiv Torques/5(rad)
  Fn in TubB/3(FzConB) -> FzConB/1, Equiv Torques/4(FzConB), Fn in SphF/4(FzConB)
  Fn in SphF/1(FySphF) -> FySphF/1
  Fn in TubB/1(FxConB) -> Equiv Torques/2(FxConB), FxConB/1, Fn in SphF/2(FxConB)
  Fn in TubB/2(FyConB) -> Equiv Torques/3(FyConB), FyConB/1, Fn in SphF/3(FyConB)
  Fn/1 -> Fn in TubB/1(Fn)
  azm/1 -> Fn in TubB/2(azm), Equiv Torques/1(azm)
  R/1 -> Fn in SphF/1(R)
  Fn in SphF/2(FxSphF) -> FxSphF/1
  Fn in SphF/3(FzSphF) -> FZSphF/1

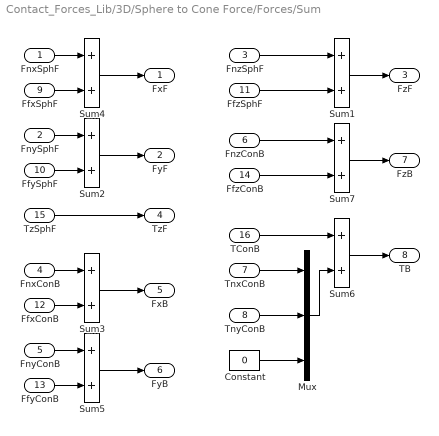
== system Contact_Forces_Lib/3D/Sphere to Cone Force/Forces/Sum ==
  FnxSphF : Inport
  FnySphF : Inport  Port=2
  FnzSphF : Inport  Port=3
  FnxConB : Inport  Port=4
  FnyConB : Inport  Port=5
  FnzConB : Inport  Port=6
  TnxConB : Inport  Port=7
  TnyConB : Inport  Port=8
  FfxSphF : Inport  Port=9
  FfySphF : Inport  Port=10
  FfzSphF : Inport  Port=11
  FfxConB : Inport  Port=12
  FfyConB : Inport  Port=13
  FfzConB : Inport  Port=14
  TzSphF : Inport  Port=15
  TConB : Inport  Port=16
  Constant : Constant  Value=0
  Mux : Mux  Inputs=3
  Sum{1..7} (7 alike) : Sum
  FxF : Outport  VectorParamsAs1DForOutWhenUnconnected=off
  FyF : Outport  Port=2  VectorParamsAs1DForOutWhenUnconnected=off
  FzF : Outport  Port=3  VectorParamsAs1DForOutWhenUnconnected=off
  TzF : Outport  Port=4  VectorParamsAs1DForOutWhenUnconnected=off
  FxB : Outport  Port=5  VectorParamsAs1DForOutWhenUnconnected=off
  FyB : Outport  Port=6  VectorParamsAs1DForOutWhenUnconnected=off
  FzB : Outport  Port=7  VectorParamsAs1DForOutWhenUnconnected=off
  TB : Outport  Port=8  VectorParamsAs1DForOutWhenUnconnected=off
  wires:
  Sum7/1 -> FzB/1
  FnzConB/1 -> Sum7/1
  Constant/1 -> Mux/3
  TnyConB/1 -> Mux/2
  TnxConB/1 -> Mux/1
  Mux/1 -> Sum6/2
  TConB/1 -> Sum6/1
  TzSphF/1 -> TzF/1
  FfyConB/1 -> Sum5/2
  FfxConB/1 -> Sum3/2
  FfySphF/1 -> Sum2/2
  FfxSphF/1 -> Sum4/2
  Sum5/1 -> FyB/1
  Sum3/1 -> FxB/1
  Sum2/1 -> FyF/1
  Sum4/1 -> FxF/1
  FnyConB/1 -> Sum5/1
  FnxConB/1 -> Sum3/1
  FnySphF/1 -> Sum2/1
  FnxSphF/1 -> Sum4/1
  Sum1/1 -> FzF/1
  FnzSphF/1 -> Sum1/1
  FfzSphF/1 -> Sum1/2
  FfzConB/1 -> Sum7/2
  Sum6/1 -> TB/1

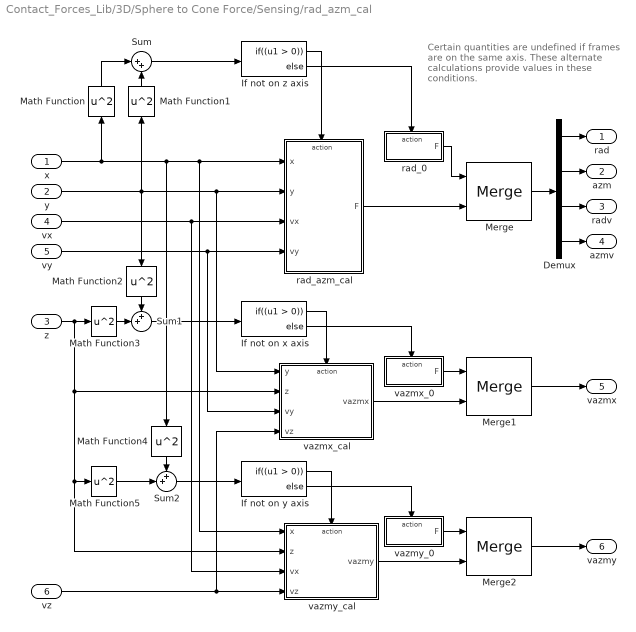
== system Contact_Forces_Lib/3D/Sphere to Cone Force/Sensing/rad_azm_cal ==
  note: Certain quantities are undefined if frames are on the same axis. These alternate calculations provide values in these conditions.
  x : Inport
  y : Inport  Port=2
  z : Inport  Port=3
  vx : Inport  Port=4
  vy : Inport  Port=5
  vz : Inport  Port=6
  Demux : Demux
  If not on x axis : If  IfExpression=(u1 > 0)
  If not on y axis : If  IfExpression=(u1 > 0)
  If not on z axis : If  IfExpression=(u1 > 0)
  Math Function{,1..5} (6 alike) : Math  Operator=square  SignedPower=on
  Merge : Merge  InitialOutput=0  InputPortOffsets=0
  Merge1 : Merge  InitialOutput=0  InputPortOffsets=0
  Merge2 : Merge  InitialOutput=0  InputPortOffsets=0
  Sum : Sum  Inputs=|++
  Sum1 : Sum  Inputs=++|
  Sum2 : Sum  Inputs=++|
  rad_0 : Subsystem
  rad_azm_cal : Subsystem
  vazmx_0 : Subsystem
  vazmx_cal : Subsystem
  vazmy_0 : Subsystem
  vazmy_cal : Subsystem
  rad : Outport  VectorParamsAs1DForOutWhenUnconnected=off
  azm : Outport  Port=2  VectorParamsAs1DForOutWhenUnconnected=off
  radv : Outport  Port=3  VectorParamsAs1DForOutWhenUnconnected=off
  azmv : Outport  Port=4  VectorParamsAs1DForOutWhenUnconnected=off
  vazmx : Outport  Port=5  VectorParamsAs1DForOutWhenUnconnected=off
  vazmy : Outport  Port=6  VectorParamsAs1DForOutWhenUnconnected=off
  wires:
  Merge2/1 -> vazmy/1
  vazmy_cal/1(vazmy) -> Merge2/2
  vazmy_0/1(F) -> Merge2/1
  Merge1/1 -> vazmx/1
  vazmx_cal/1(vazmx) -> Merge1/2
  vazmx_0/1(F) -> Merge1/1
  Sum2/1 -> If not on y axis/1
  If not on y axis/2 -> vazmy_0/Action
  If not on y axis/1 -> vazmy_cal/Action
  Math Function5/1 -> Sum2/2
  Math Function4/1 -> Sum2/1
  z/1 -> Math Function3/1, Math Function5/1, vazmy_cal/2(z), vazmx_cal/2(z)
  Sum1/1 -> If not on x axis/1
  Math Function2/1 -> Sum1/1
  Math Function3/1 -> Sum1/2
  If not on x axis/2 -> vazmx_0/Action
  If not on x axis/1 -> vazmx_cal/Action
  vz/1 -> vazmx_cal/4(vz), vazmy_cal/4(vz)
  Merge/1 -> Demux/1
  If not on z axis/1 -> rad_azm_cal/Action
  If not on z axis/2 -> rad_0/Action
  Demux/2 -> azm/1
  rad_0/1(F) -> Merge/1
  Demux/4 -> azmv/1
  Demux/1 -> rad/1
  Demux/3 -> radv/1
  vx/1 -> vazmy_cal/3(vx), rad_azm_cal/3(vx)
  x/1 -> vazmy_cal/1(x), rad_azm_cal/1(x), Math Function4/1, Math Function/1
  vy/1 -> vazmx_cal/3(vy), rad_azm_cal/4(vy)
  y/1 -> Math Function2/1, Math Function1/1, vazmx_cal/1(y), rad_azm_cal/2(y)
  rad_azm_cal/1(F) -> Merge/2
  Math Function1/1 -> Sum/2
  Math Function/1 -> Sum/1
  Sum/1 -> If not on z axis/1

== system Contact_Forces_Lib/3D/Sphere to Plane Force/Forces/Calculate Penetration ==
  z : Inport
  vz : Inport  Port=2
  Abs : Abs  ZeroCross=off  SaturateOnIntegerOverflow=off
  Constant : Constant  Value=sphere_rad+plane_depth
  Dead Zone : DeadZone  LowerValue=-inf  UpperValue=0
  Gain2 : Gain  Gain=-1
  Product : Product
  Sign vx : Signum  ZeroCross=off
  Sign x : Signum  ZeroCross=off
  Sum : Sum  Inputs=+-
  Pos Sign : Outport  VectorParamsAs1DForOutWhenUnconnected=off
  Pen : Outport  Port=2  VectorParamsAs1DForOutWhenUnconnected=off
  Pen Vel : Outport  Port=3  VectorParamsAs1DForOutWhenUnconnected=off
  Vel Sign : Outport  Port=4  VectorParamsAs1DForOutWhenUnconnected=off
  wires:
  z/1 -> Sign x/1, Abs/1
  vz/1 -> Product/2, Sign vx/1
  Constant/1 -> Sum/1
  Sum/1 -> Dead Zone/1
  Abs/1 -> Sum/2
  Sign x/1 -> Pos Sign/1, Product/1
  Sign vx/1 -> Vel Sign/1
  Product/1 -> Gain2/1
  Dead Zone/1 -> Pen/1
  Gain2/1 -> Pen Vel/1

== system Contact_Forces_Lib/3D/Sphere to Plane Force/Forces/Ff ==
  Fn : Inport
  R : Inport  Port=2
  zSign : Inport  Port=3
  wx : Inport  Port=4
  wy : Inport  Port=5
  vx : Inport  Port=6
  vy : Inport  Port=7
  Cross Product : $bdroot/Math/Cross Product  SystemSampleTime=-1  VariantActivationTime=update diagram  EmptyChoice=off  PassThrough=off  PassThroughVariantControl=(default)  EmptyChoiceVariantControl=(default)  AllowFlexibleInterface=on  Latency=0  AutoFrameSizeCalculation=off
  Friction Law : $bdroot/Friction Law  SystemSampleTime=-1  LabelModeActiveChoice=Stick_Slip_C  VariantActivationTime=update diagram  EmptyChoice=off  PassThrough=off  PassThroughVariantControl=(default)  EmptyChoiceVariantControl=(default)  AllowFlexibleInterface=on  Latency=0  AutoFrameSizeCalculation=off
  Fx1 : Constant  Value=0
  Fx2 : Constant  Value=[0 0 -sphere_rad]
  Gain : Gain  Gain=-1
  Mux1 : Mux  Inputs=3
  Product1 : Product  Inputs=/*  Multiplication=Matrix(*)
  Product2 : Product  Inputs=/*  Multiplication=Matrix(*)
  Product{3..7} (5 alike) : Product
  Selector : Selector  InputPortWidth=3  IndexOptions=Index vector (dialog)  Indices=3  OutputSizes=1
  SlipVel : Subsystem
  Trigonometric Function : Trigonometry
  Trigonometric Function1 : Trigonometry  Operator=cos
  zSign1 : InportShadow  Port=3
  Ff Sph : Outport  VectorParamsAs1DForOutWhenUnconnected=off
  T Sph : Outport  Port=2  VectorParamsAs1DForOutWhenUnconnected=off
  Ff Pla : Outport  Port=3  VectorParamsAs1DForOutWhenUnconnected=off
  wires:
  Fn/1 -> Selector/1
  Gain/1 -> Ff Pla/1
  SlipVel/2(alpha) -> Trigonometric Function/1, Trigonometric Function1/1
  Trigonometric Function1/1 -> Product3/2
  SlipVel/1(vabs) -> Friction Law/2
  Selector/1 -> Friction Law/1
  Friction Law/1 -> Product3/1, Product4/1
  Product4/1 -> Mux1/2
  Product3/1 -> Mux1/1
  Fx1/1 -> Mux1/3
  Trigonometric Function/1 -> Product4/2
  vx/1 -> Product6/1
  wx/1 -> SlipVel/1(wx)
  wy/1 -> SlipVel/2(wy)
  vy/1 -> Product5/2
  Product2/1 -> T Sph/1
  Mux1/1 -> Gain/1, Cross Product/2, Product1/2
  Product1/1 -> Ff Sph/1
  Cross Product/1 -> Product2/2
  R/1 -> Product1/1, Product2/1
  Fx2/1 -> Product7/1
  Product5/1 -> SlipVel/4(vy)
  zSign/1 -> Product5/1, Product6/2
  Product6/1 -> SlipVel/3(vx)
  zSign1/1 -> Product7/2
  Product7/1 -> Cross Product/1

== system Contact_Forces_Lib/3D/Sphere to Plane Force/Forces/Fn ==
  R : Inport
  SprF : Inport  Port=2
  DamF : Inport  Port=3
  Fx : Constant  Value=0
  Gain : Gain  Gain=-1
  Mux : Mux  Inputs=3
  Product2 : Product  Inputs=/*  Multiplication=Matrix(*)
  Sum : Sum
  Fn : Outport  VectorParamsAs1DForOutWhenUnconnected=off
  FnF : Outport  Port=2  VectorParamsAs1DForOutWhenUnconnected=off
  FnB : Outport  Port=3  VectorParamsAs1DForOutWhenUnconnected=off
  wires:
  Mux/1 -> Gain/1, Product2/2
  Product2/1 -> FnF/1
  Gain/1 -> FnB/1
  R/1 -> Product2/1
  Fx/1 -> Mux/1, Mux/2
  Sum/1 -> Fn/1, Mux/3
  DamF/1 -> Sum/2
  SprF/1 -> Sum/1

== system Contact_Forces_Lib/3D/Sphere to Plane Force Enabled/Forces/Calculate Penetration ==
  z : Inport
  vz : Inport  Port=2
  Abs : Abs  ZeroCross=off  SaturateOnIntegerOverflow=off
  Constant : Constant  Value=sphere_rad+plane_depth
  Dead Zone : DeadZone  LowerValue=-inf  UpperValue=0
  Gain2 : Gain  Gain=-1
  Product : Product
  Sign vx : Signum  ZeroCross=off
  Sign x : Signum  ZeroCross=off
  Sum : Sum  Inputs=+-
  Pos Sign : Outport  VectorParamsAs1DForOutWhenUnconnected=off
  Pen : Outport  Port=2  VectorParamsAs1DForOutWhenUnconnected=off
  Pen Vel : Outport  Port=3  VectorParamsAs1DForOutWhenUnconnected=off
  Vel Sign : Outport  Port=4  VectorParamsAs1DForOutWhenUnconnected=off
  wires:
  Gain2/1 -> Pen Vel/1
  Dead Zone/1 -> Pen/1
  Product/1 -> Gain2/1
  Sign vx/1 -> Vel Sign/1
  Sign x/1 -> Product/1, Pos Sign/1
  Abs/1 -> Sum/2
  Sum/1 -> Dead Zone/1
  Constant/1 -> Sum/1
  vz/1 -> Sign vx/1, Product/2
  z/1 -> Abs/1, Sign x/1
